simulink model "gtm_design"  (R2021b)
settings: Solver=VariableStepAuto  StartTime=0.0  StopTime=10.0  MinStep=0.00999  RelTol=1e-3
StopFcn:
  | MWSout=grabmws(bdroot);
  | MWSout.lastrun=datestr(now);
values from neighbouring files (symbols this model uses):
  knots2fps = 1.68781    [setup.m]
  s = tf('s')    [setup.m]
undefined symbols (not defined in the file or in its folder): Aero, aftfuel, aftfuel_pos, AILL, AILLC, AILR, AILRC, alpha_deg, alt0, altitude_ft, Ax_g, Ay_g, Az_g, b, beta_deg, bias, BRAKEC, Cbar, cg_pos0, cg_shift_gear, ControlMode, DamageCase, DamageModels, DamageOnsetTime, deltc, Earth, ELLIB, ELLIBC, ELLOB, ELLOBC, ELRIB, ELRIBC, ELROB, ELROBC, engl_ang, engl_pos, engr_ang, engr_pos, etas0, etas1, etasc_feedthrough, FLAPLC, FLAPLIB, FLAPLOB, FLAPRC, FLAPRIB, FLAPROB, FlightMode, FuelUsed_Init, fwdfuel, fwdfuel_pos, GEAR, GEARC, Inertia0, Inertia_shift_gear, Ixx_model, Iyy_model, Izz_model, KTAS, LandingGear ... (+66)
libraries: simulink_extras x98, LPVBlockLibrary x54, simulink_need_slupdate x30, aerolibconvert2 x27, simulink x7, aerolibtransform2 x6, uavalgslib x4, UserContent_lib x2, robotcorelib x1, uavutilslib x1
(part 2 of 9)

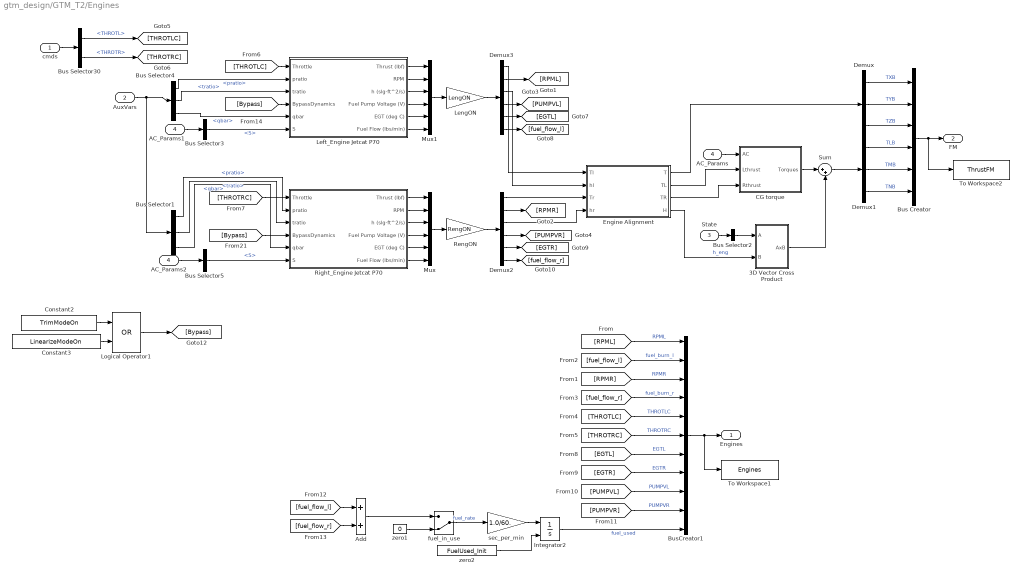
== system gtm_design/GTM_T2/Engines ==
  cmds : Inport
  AuxVars : Inport  Port=2
  State : Inport  Port=3
  AC_Params : Inport  Port=4
  3D Vector Cross Product : Subsystem
  AC_Params1 : InportShadow  Port=4
  AC_Params2 : InportShadow  Port=4
  Add : Sum
  Bus Creator : BusCreator  Inputs=6
  Bus Selector1 : BusSelector  OutputSignals=pratio,tratio,qbar
  Bus Selector2 : BusSelector  OutputSignals=pb,qb,rb  OutputAsBus=on
  Bus Selector3 : BusSelector  OutputSignals=S
  Bus Selector30 : BusSelector  OutputSignals=THROTL,THROTR
  Bus Selector4 : BusSelector  OutputSignals=pratio,tratio,qbar
  Bus Selector5 : BusSelector  OutputSignals=S
  BusCreator1 : BusCreator  Inputs=11
  CG torque : Subsystem
  Constant2 : Constant  Value=TrimModeOn
  Constant3 : Constant  Value=LinearizeModeOn
  Demux : Demux  Outputs=3
  Demux1 : Demux  Outputs=3
  Demux2 : Demux  Outputs=6
  Demux3 : Demux  Outputs=6
  Engine Alignment : MATLAB Function  TreatAsAtomicUnit=on
  Integrator2 : Integrator  InitialConditionSource=external
  Left_Engine Jetcat P70 : Subsystem
      mask init:
      | % Curve fit parameters for Jetcat P70 Model
      | % Coeff_thrust   = [0.000028864242464  -0.001914835880159 0.105916926095459  -1.251646340183624 ];
      | Coeff_thrust   = [0.000014847593013,  0, 0, 0.412662356277121];
      | Coeff_throttle = [0.000033035538475  -0.008354385314499 1.191126728328792 31.518959847101669];
      | Coeff_fuelflow = [0.000046800927870  -0.000779344124807 0.122178501497750];
      | Coeff_tau      = [ -2.2400e-02   2.9948e+00];
      | Coeff_EGT      = [ 2E-5, -0.0036,0.2342,-8.0496,664.99]; %EGT model, deg C
      | Coeff_dynamics = [ -.074 7.1];
      | fuelpump_table = [0 0.576	0.625	0.6985	0.7845	0.8575	0.919	0.9805	1.0415	1.1025...
      |                     1.1515	1.262	1.287	1.373	1.52	1.618	1.74	1.887	1.973...
      |                     2.12	2.255	2.4385	2.647	2.7575	2.9905	3.162]; %volts, table of fuel pump voltages
      | fuelflow_table = [0,0.0794,0.0876,0.102,0.1149,0.1275,0.1379,0.1487,0.1586,0.1671,...
      |                     0.1775,0.1858,0.194,0.2038,0.2206,0.2405,0.2566,0.2746,0.2921,0.3102,...
      |                     0.3266,0.3445,0.3533,0.3611,0.3866,0.4083;]*2; %lbs/min,   FULL fuel flow rates corresponding to pump voltages (fuelpump_table)  
      | % Equvalent Shaft parameters for engine
      | shaft_dia = 0.75/12.0;       % diameter of rotating turbine in feet 
      | shaft_len = 6.25/12.0;       % length of rotating turbine in feet   
      | density   = 15.2;            % mass density of steel in slugs/ft^3 
      | 
      | 
      | A = [-1.336,-0.7314;1,0;];
      | B = [1;0];
      | C = [-0.1474   0.7314];
      | D = 0;
  LengON : Gain  Gain=LengON  SaturateOnIntegerOverflow=on  OutDataTypeStr=Inherit: Same as input  ParamDataTypeStr=Inherit: Same as input
  Logical Operator1 : Logic  Operator=OR  AllPortsSameDT=off  OutDataTypeStr=boolean
  Mux : Mux  Inputs=6
  Mux1 : Mux  Inputs=6
  RengON : Gain  Gain=RengON  SaturateOnIntegerOverflow=on  OutDataTypeStr=Inherit: Same as input  ParamDataTypeStr=Inherit: Same as input
  Right_Engine Jetcat P70 : Subsystem
      mask init: same as gtm_design/GTM_T2/Engines/Left_Engine Jetcat P70
  Sum : Sum  Inputs=|++
  To Workspace1 : ToWorkspace  VariableName=Engines  SampleTime=-1
  To Workspace2 : ToWorkspace  VariableName=ThrustFM  SampleTime=-1
  fuel_in_use : ManualSwitch  CurrentSetting=0
  sec_per_min : Gain  Gain=1.0/60.  SaturateOnIntegerOverflow=on  OutDataTypeStr=Inherit: Same as input  ParamDataTypeStr=Inherit: Same as input
  zero1 : Constant  Value=0
  zero2 : Constant  Value=FuelUsed_Init
  Engines : Outport
  FM : Outport  Port=2  PortDimensions=6
  wires:
  cmds/1 -> Bus Selector30/1
  Demux/2 -> Bus Creator/2  "TYB"
  State/1 -> Bus Selector2/1
  Bus Selector2/1 -> 3D Vector Cross Product/1(A)
  Demux/3 -> Bus Creator/3  "TZB"
  AuxVars/1 -> Bus Selector1/1, Bus Selector4/1
  AC_Params/1 -> CG torque/1(AC)
  Bus Creator/1 -> To Workspace2/1, FM/1
  Bus Selector30/1 -> [THROTLC]  "<THROTL>"
  Bus Selector30/2 -> [THROTRC]  "<THROTR>"
  [THROTRC] -> BusCreator1/6  "THROTRC"
  [THROTLC] -> BusCreator1/5  "THROTLC"
  [fuel_flow_r] -> BusCreator1/4  "fuel_burn_r"
  [fuel_flow_l] -> BusCreator1/2  "fuel_burn_l"
  [RPMR] -> BusCreator1/3  "RPMR"
  [RPML] -> BusCreator1/1  "RPML"
  BusCreator1/1 -> To Workspace1/1, Engines/1
  [EGTL] -> BusCreator1/7  "EGTL"
  [EGTR] -> BusCreator1/8  "EGTR"
  [PUMPVL] -> BusCreator1/9  "PUMPVL"
  [PUMPVR] -> BusCreator1/10  "PUMPVR"
  sec_per_min/1 -> Integrator2/1
  fuel_in_use/1 -> sec_per_min/1  "fuel_rate"
  Integrator2/1 -> BusCreator1/11  "fuel_used"
  zero2/1 -> Integrator2/2
  [fuel_flow_l] -> Add/1
  [fuel_flow_r] -> Add/2
  zero1/1 -> fuel_in_use/2
  Add/1 -> fuel_in_use/1
  Demux/1 -> Bus Creator/1  "TXB"
  Engine Alignment/4(H) -> 3D Vector Cross Product/2(B)  "h_eng"
  Engine Alignment/1(T) -> Demux/1
  Engine Alignment/2(TL) -> CG torque/2(Lthrust)
  Engine Alignment/3(TR) -> CG torque/3(Rthrust)
  CG torque/1(Torques) -> Sum/1
  3D Vector Cross Product/1(AxB) -> Sum/2
  Sum/1 -> Demux1/1
  Demux1/1 -> Bus Creator/4  "TLB"
  Demux1/2 -> Bus Creator/5  "TMB"
  Demux1/3 -> Bus Creator/6  "TNB"
  Mux/1 -> RengON/1
  RengON/1 -> Demux2/1
  Demux2/1 -> Engine Alignment/3(Tr)
  Demux2/2 -> [RPMR]
  Demux2/3 -> Engine Alignment/4(hr)
  Demux2/4 -> [PUMPVR]
  Demux2/5 -> [EGTR]
  Demux2/6 -> [fuel_flow_r]
  Mux1/1 -> LengON/1
  LengON/1 -> Demux3/1
  Demux3/1 -> Engine Alignment/1(Tl)
  Demux3/2 -> [RPML]
  Demux3/3 -> Engine Alignment/2(hl)
  Demux3/4 -> [PUMPVL]
  Demux3/5 -> [EGTL]
  Demux3/6 -> [fuel_flow_l]
  Constant3/1 -> Logical Operator1/2
  Constant2/1 -> Logical Operator1/1
  Logical Operator1/1 -> [Bypass]
  Left_Engine Jetcat P70/1(Thrust (lbf)) -> Mux1/1
  Left_Engine Jetcat P70/2(RPM) -> Mux1/2
  Left_Engine Jetcat P70/3(h (slg-ft^2/s)) -> Mux1/3
  Left_Engine Jetcat P70/4(Fuel Pump Voltage (V)) -> Mux1/4
  Left_Engine Jetcat P70/5(EGT (deg C)) -> Mux1/5
  Left_Engine Jetcat P70/6(Fuel Flow (lbs/min)) -> Mux1/6
  Right_Engine Jetcat P70/1(Thrust (lbf)) -> Mux/1
  Right_Engine Jetcat P70/2(RPM) -> Mux/2
  Right_Engine Jetcat P70/3(h (slg-ft^2/s)) -> Mux/3
  Right_Engine Jetcat P70/4(Fuel Pump Voltage (V)) -> Mux/4
  Right_Engine Jetcat P70/5(EGT (deg C)) -> Mux/5
  Right_Engine Jetcat P70/6(Fuel Flow (lbs/min)) -> Mux/6
  AC_Params2/1 -> Bus Selector5/1
  AC_Params1/1 -> Bus Selector3/1
  [THROTRC] -> Right_Engine Jetcat P70/1(Throttle)
  Bus Selector4/1 -> Left_Engine Jetcat P70/2(pratio)  "<pratio>"
  Bus Selector4/2 -> Left_Engine Jetcat P70/3(tratio)  "<tratio>"
  [Bypass] -> Left_Engine Jetcat P70/4(BypassDynamics)
  Bus Selector4/3 -> Left_Engine Jetcat P70/5(qbar)  "<qbar>"
  Bus Selector3/1 -> Left_Engine Jetcat P70/6(S)  "<S>"
  Bus Selector1/1 -> Right_Engine Jetcat P70/2(pratio)  "<pratio>"
  Bus Selector1/2 -> Right_Engine Jetcat P70/3(tratio)  "<tratio>"
  [Bypass] -> Right_Engine Jetcat P70/4(BypassDynamics)
  Bus Selector1/3 -> Right_Engine Jetcat P70/5(qbar)  "<qbar>"
  Bus Selector5/1 -> Right_Engine Jetcat P70/6(S)  "<S>"
  [THROTLC] -> Left_Engine Jetcat P70/1(Throttle)

== system gtm_design/GTM_T2/Gravity ==
  AuxVars : Inport
  Params : Inport  Port=2
  Bus Selector1 : BusSelector  OutputSignals=DCM
  Bus Selector6 : BusSelector  OutputSignals=mass
  Ground : Ground
  Ground1 : Ground
  Mux : Mux  Inputs=[3 3]
  Mux1 : Mux  Inputs=3
  Product : Product  Multiplication=Matrix(*)  RndMeth=Zero
  Product1 : Product  RndMeth=Zero
  To Workspace2 : ToWorkspace  VariableName=GravityFM  SampleTime=-1
  acc due to gravity (ft/s^2) : Constant  Value=32.17405
  FM : Outport
  wires:
  acc due to gravity (ft/s^2)/1 -> Product1/2
  Ground1/1 -> Mux/2
  Product1/1 -> Mux1/3
  Ground/1 -> Mux1/2, Mux1/1
  Mux1/1 -> Product/2
  Mux/1 -> To Workspace2/1, FM/1
  Product/1 -> Mux/1
  Params/1 -> Bus Selector6/1
  AuxVars/1 -> Bus Selector1/1
  Bus Selector1/1 -> Product/1  "<DCM>"
  Bus Selector6/1 -> Product1/1  "<mass>"

== system gtm_design/GTM_T2/Landing Gear ==
  State : Inport
  Surfaces : Inport  Port=2
  ACParams : Inport  Port=3
  Bus Selector : BusSelector  OutputSignals=BRAKE,STEER,GEAR
  Bus Selector1 : BusSelector  OutputSignals=pb,qb,rb  OutputAsBus=on
  Bus Selector2 : BusSelector  OutputSignals=ub,vb,wb  OutputAsBus=on
  Bus Selector3 : BusSelector  OutputSignals=psi
  Bus Selector4 : BusSelector  OutputSignals=altitude
  Bus Selector5 : BusSelector  OutputSignals=phi,theta,psi  OutputAsBus=on
  Bus Selector6 : BusSelector  OutputSignals=CG  OutputAsBus=on
  Bus to Vector : BusToVector
  Bus to Vector1 : BusToVector
  Bus to Vector2 : BusToVector
  Gain : Gain  Gain=1/100
  LandingGear : Subsystem  mask{NoseWheelPos=LandingGear.NoseWheelPos, LeftMainPos=LandingGear.LeftMainPos, RightMainPos=LandingGear.RightMainPos, SpringConst=LandingGear.SpringConst, DampingConst=LandingGear.DampingConst, StrokeLength=LandingGear.StrokeLength, MountStiffness=LandingGear.MountStiff, MountDamping=LandingGear.MountDamping, RunwayAlt=runway_alt}
      mask prompts: NoseWheelPos "Nose Wheel Position [X,Y,Z]"; LeftMainPos "Left Main Position [X,Y,Z]"; RightMainPos "Right Main Position [X,Y,Z]"; SpringConst "Spring Constant [Nose,Left,Right]"; DampingConst "Damping Constant [Nose,Left,Right]"; StrokeLength "Stroke Length [Nose,Left,Right]"; MountStiffness "Mount Stiffness [Nose,Left,Right]"; MountDamping "Mount Damping [Nose,Left, Right]"; RunwayAlt "Runway Altitude"
      mask help:
      | Implements ground reaction force (if geardown is nonzero) for 3-wheel landing gear. Linear stiffness and damping are applied within stroke range, and (generally larger) mount stiffness and damping are applied beyond this range.
      |
      | Underlying gear.c function is from HL-20/LaRCsim, e.b.jackson@nasa.gov
  Mux : Mux  Inputs=2
  To Workspace1 : ToWorkspace  VariableName=GearState  SampleTime=-1
  To Workspace2 : ToWorkspace  VariableName=GearFM  SampleTime=-1
  FM : Outport
  GearState : Outport  Port=2
  wires:
  Mux/1 -> To Workspace2/1, FM/1
  Gain/1 -> LandingGear/7(Brake (0-1))
  LandingGear/3(Contact) -> To Workspace1/1, GearState/1
  LandingGear/2(M_gear) -> Mux/2
  LandingGear/1(F_gear) -> Mux/1
  Bus Selector/3 -> LandingGear/9(geardown (0/1))  "<GEAR>"
  Bus Selector/2 -> LandingGear/8(Steer (deg))  "<STEER>"
  Bus Selector/1 -> Gain/1  "<BRAKE>"
  Bus Selector3/1 -> LandingGear/6(Heading (Rad))  "<psi>"
  Bus to Vector/1 -> LandingGear/4(pqr (Rad/sec))
  Bus Selector4/1 -> LandingGear/3(Altitude (ft))  "<altitude>"
  Bus to Vector2/1 -> LandingGear/2(EulerAngles (Rad))
  Bus Selector6/1 -> LandingGear/1(cg)
  Surfaces/1 -> Bus Selector/1
  State/1 -> Bus Selector1/1, Bus Selector2/1, Bus Selector3/1, Bus Selector4/1, Bus Selector5/1
  Bus Selector1/1 -> Bus to Vector/1
  Bus to Vector1/1 -> LandingGear/5(Vbody (ft/sec))
  Bus Selector2/1 -> Bus to Vector1/1
  Bus Selector5/1 -> Bus to Vector2/1
  ACParams/1 -> Bus Selector6/1

== system gtm_design/GTM_T2/Sensors ==
  EOM_State : Inport
  EOM_Xdot : Inport  Port=2
  AC_Params : Inport  Port=3
  AuxVars : Inport  Port=4
  SurfacePos : Inport  Port=5
  Engines : Inport  Port=6
  Air Data : Subsystem
  AuxVars1 : InportShadow  Port=4
  Bus Creator : BusCreator  Inputs=5
  Engine ECU 8 Hz : Subsystem  SystemSampleTime=round(1/Timestep/8)*Timestep
  MAG3 IMU : Subsystem
  MIDG II 50 Hz : Subsystem  SystemSampleTime=round(1/Timestep/50)*Timestep
  Surface Pots : Subsystem
  Terminator : Terminator
  Terminator1 : Terminator
  To Workspace2 : ToWorkspace  VariableName=Sensors  SampleTime=-1
  Sensors : Outport
  wires:
  AC_Params/1 -> Terminator1/1
  EOM_Xdot/1 -> Terminator/1
  Bus Creator/1 -> To Workspace2/1, Sensors/1
  Air Data/1(AirData) -> Bus Creator/1  "AirData"
  MIDG II 50 Hz/1(MIDG) -> Bus Creator/2  "MIDG"
  Surface Pots/1(Pots) -> Bus Creator/4  "SurfacePos"
  Engine ECU 8 Hz/1(ECU) -> Bus Creator/5  "Engines"
  MAG3 IMU/1(MAG3) -> Bus Creator/3  "MAG3"
  Engines/1 -> Engine ECU 8 Hz/1(Engines)
  SurfacePos/1 -> Surface Pots/1(SurfacePos)
  AuxVars/1 -> Air Data/2(AuxVars), MIDG II 50 Hz/1(AuxVars)
  EOM_State/1 -> MIDG II 50 Hz/2(EOM_State), Air Data/1(EOM_State), MAG3 IMU/2(EOM_State)
  AuxVars1/1 -> MAG3 IMU/1(AuxVars)

== system gtm_design/GTM_T2/TransportDelay ==
  note: Uplink Path
  note: Downlink Path
  Sensors : Inport
  UL : Inport  Port=2
  AntiAliasing : Subsystem
  To Workspace2 : ToWorkspace  VariableName=DL  SampleTime=-1
  Transport Delay on Bus : Subsystem
  Transport Delay on Bus1 : Subsystem
  cmds : Outport
  DL : Outport  Port=2
  wires:
  AntiAliasing/1(O) -> Transport Delay on Bus/1(In)
  Transport Delay on Bus/1(Out) -> To Workspace2/1, DL/1
  UL/1 -> Transport Delay on Bus1/1(In)
  Sensors/1 -> AntiAliasing/1(I)
  Transport Delay on Bus1/1(Out) -> cmds/1

== system gtm_design/Guidance/Airspeed Step ==
  Action Port : ActionPort  ActionPortLabel=case [ 3 ]:
  Bus Creator : BusCreator  Inputs=5
  Constant1 : Constant  Value=-12.5
  Constant2 : Constant  Value=0
  Constant3 : Constant  Value=0
  Constant4 : Constant  Value=0
  Step : Step  Time=5  Before=80  After=90  SampleTime=0
  Step1 : Step  Commented=on  Time=50  After=-5  SampleTime=0
  Sum : Sum  Inputs=|++
  GuidanceCommand : Outport  InitialOutput=zeros(5,1)
  wires:
  Constant2/1 -> Bus Creator/2  "alt_c_ft"
  Constant4/1 -> Bus Creator/4  "phi_c_deg"
  Bus Creator/1 -> GuidanceCommand/1
  Constant3/1 -> Bus Creator/3  "bet_c_deg"
  Sum/1 -> Bus Creator/1  "tas_c_knot"
  Constant1/1 -> Bus Creator/5  "etas_c_percent"
  Step/1 -> Sum/1
  Step1/1 -> Sum/2

== system gtm_design/Guidance/Autopilot Step ==
  Action Port : ActionPort  ActionPortLabel=case [ 3 ]:
  Airspeed Step Command : Subsystem
  Altitude Step Command : Subsystem
  Constant : Constant  Value=3
  Gain : Gain  Gain=10
  GuidanceMode1 : Constant  Value=FlightMode
  Label : Subsystem
  Merge1 : Merge  Inputs=5
  Roll Angle Step Command : Subsystem
  Sideslip Step Command : Subsystem
  Sum : Sum  Inputs=|+-
  Switch Case1 : SwitchCase  CaseConditions={1,2,3,4}
  Zero : Subsystem
  round : Rounding  Operator=round
  cmd : Outport
  wires:
  Label/1(O) -> cmd/1
  Merge1/1 -> Label/1(I)
  Switch Case1/5 -> Zero/Action  "FlightMode == 3.0"
  Switch Case1/3 -> Sideslip Step Command/Action  "FlightMode == 3.3"
  Switch Case1/2 -> Altitude Step Command/Action  "FlightMode == 3.2"
  Switch Case1/1 -> Airspeed Step Command/Action  "FlightMode == 3.1"
  Sideslip Step Command/1(cmd) -> Merge1/3
  Airspeed Step Command/1(cmd) -> Merge1/1
  Altitude Step Command/1(cmd) -> Merge1/2
  Gain/1 -> round/1
  Sum/1 -> Gain/1
  Constant/1 -> Sum/2
  GuidanceMode1/1 -> Sum/1
  Roll Angle Step Command/1(cmd) -> Merge1/4
  Zero/1(cmd) -> Merge1/5
  Switch Case1/4 -> Roll Angle Step Command/Action  "FlightMode == 3.4"
  round/1 -> Switch Case1/1

== system gtm_design/Guidance/Autopilot Trajectory Tracking ==
  feedback : Inport
  Action Port : ActionPort  ActionPortLabel=case [ 4 ]:
  Constant : Constant  Value=4
  Constant1 : Constant  Value=4
  Constant2 : Constant  Value=2
  Gain : Gain  Gain=10
  Gain1 : Gain  Gain=10
  GuidanceMode1 : Constant  Value=FlightMode
  GuidanceMode2 : Constant  Value=FlightMode
  Label : Subsystem
  Orbit Following : Subsystem
  Sum : Sum  Inputs=|+-
  Sum1 : Sum  Inputs=|+-
  Sum2 : Sum  Inputs=|-+
  Switch : Switch  Criteria=u2 ~= 0
  Switch Case1 : SwitchCase  CaseConditions={1,2}  ShowDefaultCase=off
  Waypoint Following : Subsystem
  feedback1 : InportShadow
  round : Rounding  Operator=round
  round1 : Rounding  Operator=round
  guidance_cmd : Outport
  wires:
  Constant/1 -> Sum/2
  GuidanceMode1/1 -> Sum/1
  Waypoint Following/1(guidance_cmd) -> Switch/1
  Label/1(O) -> guidance_cmd/1
  Switch Case1/1 -> Waypoint Following/Action  "FlightMode == 4.1"
  Switch Case1/2 -> Orbit Following/Action  "FlightMode == 4.2"
  Sum/1 -> Gain/1
  Gain/1 -> round/1
  Orbit Following/1(guidance_cmd) -> Switch/3
  feedback/1 -> Waypoint Following/1(Feedback)
  feedback1/1 -> Orbit Following/1(Feedback)
  round/1 -> Switch Case1/1
  Sum1/1 -> Gain1/1
  GuidanceMode2/1 -> Sum1/1
  Gain1/1 -> round1/1
  Constant1/1 -> Sum1/2
  round1/1 -> Sum2/1
  Constant2/1 -> Sum2/2
  Sum2/1 -> Switch/2
  Switch/1 -> Label/1(I)

== system gtm_design/Guidance/CAS Maneuver ==
  Action Port : ActionPort  ActionPortLabel=case [ 2 ]:
  Constant : Constant  Value=2
  Gain : Gain  Gain=10
  GuidanceMode1 : Constant  Value=FlightMode
  High-g Turn : Subsystem
  Label : Subsystem
  Merge1 : Merge
  Push-over and Pull-up : Subsystem  Commented=on
  Sum : Sum  Inputs=|+-
  Switch Case1 : SwitchCase  CaseConditions={1,2}  ShowDefaultCase=off
  round : Rounding  Operator=round
  cmd : Outport
  wires:
  Label/1(O) -> cmd/1
  Merge1/1 -> Label/1(I)
  Switch Case1/2 -> High-g Turn/Action  "FlightMode == 2.2"
  Switch Case1/1 -> Push-over and Pull-up/Action  "FlightMode == 2.1"
  Gain/1 -> round/1
  Sum/1 -> Gain/1
  Constant/1 -> Sum/2
  GuidanceMode1/1 -> Sum/1
  Push-over and Pull-up/1(Out1) -> Merge1/1
  High-g Turn/1(Out1) -> Merge1/2
  round/1 -> Switch Case1/1

== system gtm_design/Guidance/CAS Step ==
  Action Port : ActionPort  ActionPortLabel=case [ 1 ]:
  Constant : Constant
  Gain : Gain  Gain=10
  GuidanceMode1 : Constant  Value=FlightMode
  Label : Subsystem
  Merge1 : Merge  Inputs=4
  Normal Acceleration Step Command : Subsystem
  Roll Rate Step Command : Subsystem
  Sideslip Step Command : Subsystem
  Sum : Sum  Inputs=|+-
  Switch Case1 : SwitchCase  CaseConditions={1,2,3}
  Zero : Subsystem
  round : Rounding  Operator=round
  cmd : Outport
  wires:
  GuidanceMode1/1 -> Sum/1
  Constant/1 -> Sum/2
  Sum/1 -> Gain/1
  Gain/1 -> round/1
  Sideslip Step Command/1(cmd) -> Merge1/2
  Normal Acceleration Step Command/1(cmd) -> Merge1/1
  Zero/1(cmd) -> Merge1/4
  Roll Rate Step Command/1(cmd) -> Merge1/3
  Switch Case1/1 -> Normal Acceleration Step Command/Action  "FlightMode == 1.1"
  Switch Case1/2 -> Sideslip Step Command/Action  "FlightMode == 1.2"
  Switch Case1/3 -> Roll Rate Step Command/Action  "FlightMode == 1.3"
  Switch Case1/4 -> Zero/Action  "FlightMode == 1.0"
  Merge1/1 -> Label/1(I)
  Label/1(O) -> cmd/1
  round/1 -> Switch Case1/1

== system gtm_design/Guidance/Elevation Step ==
  Action Port : ActionPort  ActionPortLabel=case [ 2 ]:
  Bus Creator : BusCreator  Inputs=5
  Constant : Constant  Value=80
  Constant1 : Constant  Value=-12.5
  Constant3 : Constant  Value=0
  Constant4 : Constant  Value=0
  Step : Step  After=10  SampleTime=0
  Step1 : Step  Commented=on  Time=50  After=-10  SampleTime=0
  Sum : Sum  Inputs=|++
  GuidanceCommand : Outport  InitialOutput=zeros(5,1)
  wires:
  Constant/1 -> Bus Creator/1  "tas_c_knot"
  Constant1/1 -> Bus Creator/5  "etas_c_percent"
  Constant3/1 -> Bus Creator/3  "bet_c_deg"
  Constant4/1 -> Bus Creator/4  "phi_c_deg"
  Bus Creator/1 -> GuidanceCommand/1
  Sum/1 -> Bus Creator/2  "alt_c_ft"
  Step1/1 -> Sum/2
  Step/1 -> Sum/1

== system gtm_design/Guidance/Heading Control ==
  guidance_cmd : Inport
  Feedback : Inport  Port=2
  Bus Creator1 : BusCreator  Inputs=7
  Bus Selector : BusSelector  OutputSignals=signal11
  Bus Selector1 : BusSelector  OutputSignals=alt_c_ft
  Constant1 : Constant  Value=tas0
  Constant3 : Constant  Value=0
  Constant4 : Constant  Value=0
  Constant5 : Constant  Value=etas0
  Constant6 : Constant
  FlightState : Subsystem
  Heading Control : MATLAB Function  TreatAsAtomicUnit=on  mask(Fixed Wing Heading Controller){PHeadingAngle=3.9}
      mask prompts: PHeadingAngle "Heading Control Gain"
      mask help: P controller that regulates fixed wing UAV heading direction through controlling its roll angle. This controller requires that the plane is flying under coordinated flight condition.
  Radians to Degrees : simulink_extras/Transformations/Radians to Degrees
  Saturation : Saturate  UpperLimit=phi_lim  LowerLimit=-phi_lim
  Windless : Subsystem  VariantControl=NoWind
      settings: PortSchema="{\"entries\":[{\"content\":{\"sides\":[{\"content\":{\"connectorIds\":[\"Out1\"]},\"type\":\"ConnectorPlacement.EquallySpacedRectSide\",\"uuid\":\"203a2d2a-30ae-46d5-b636-10933e29d1fa\"},{\"content\":{\"connectorIds\":[],\"side\":\"RIGHT\"},\"type\":\"ConnectorPlacement.EquallySpacedRectSide\",\"uuid\":\"332a648b-f7fb-47c3-be36-01d9c1955b3b\"},{\"content\":{\"connectorIds\":[],\"side\":\"TOP\"},\"type\":\"ConnectorPlacement.EquallySpacedRectSide\",\"uuid\":\"0294cf6c-fac0-4906-9702-b8e9ef362c1f\"}]},\"type\":\"ConnectorPlacement.EquallySpacedConnector\",\"uuid\":\"f608bdaf-466f-4a8f-9e8f-8d2734bc1053\"}],\"packageUris\":[\"http://schema.mathworks.com/mf0/Connector/R2020b\"],\"version\":\"1.0\"}"
  cmd : Outport
  wires:
  Radians to Degrees/1 -> Saturation/1
  Heading Control/1(RollAngle) -> Radians to Degrees/1  "phi_c_rad"
  Windless/1(Environment) -> Heading Control/3(e)
  Feedback/1 -> FlightState/1(Feedback)
  FlightState/1(FlightState) -> Heading Control/1(FlightState)  "FlightState"
  guidance_cmd/1 -> Bus Selector/1, Bus Selector1/1
  Bus Selector/1 -> Heading Control/2(UHeading)  "<signal11>"
  Bus Selector1/1 -> Bus Creator1/2  "<alt_c_ft>"
  Constant3/1 -> Bus Creator1/3  "bet_c_deg"
  Constant1/1 -> Bus Creator1/1  "tas_c_knot"
  Constant6/1 -> Bus Creator1/5  "an_c_g"
  Constant5/1 -> Bus Creator1/7  "etas_c_percent"
  Saturation/1 -> Bus Creator1/4  "phi_c_deg"
  Constant4/1 -> Bus Creator1/6  "p_c_deg"
  Bus Creator1/1 -> cmd/1

== system gtm_design/Guidance/Invalid, Error Out ==
  Action Port : ActionPort  ActionPortLabel=default:
  Constant1 : Constant  Value=zeros(5,1)
  Constant2 : Constant  Value=0
  InvalidMode : Assertion  AssertionFailFcn="warndlg('Invalid settings for TrimMode and LinearizeMode.  Run setup.m to reset.','Warning!')"
  Out : Outport  InitialOutput=zeros(5,1)
  wires:
  Constant1/1 -> Out/1
  Constant2/1 -> InvalidMode/1

== system gtm_design/Guidance/Label ==
  I : Inport
  I1 : Inport  Port=2
  Abs : Abs
  Add : Sum  Inputs=+++
  Bus Creator1 : BusCreator  Inputs=7
  Bus Selector : BusSelector  Commented=on  OutputSignals=AirData.KTAS,MIDG.NAV_altitude_m
  Demux1 : Demux  Outputs=7
  Gain : Gain  Gain=phi_to_eta
  Length Conversion : aerolibconvert2/Length Conversion  Commented=on  IU=m  OU=ft
  MATLAB Function : MATLAB Function  Commented=on  TreatAsAtomicUnit=on
  MATLAB Function1 : MATLAB Function  Commented=on  TreatAsAtomicUnit=on
  Ramp : simulink/Sources/Ramp  slope=RateofClimb  start=20  InitialOutput=0
  Ramp1 : simulink/Sources/Ramp  Commented=on  slope=0.1  start=0  InitialOutput=0
  Sum : Sum  Inputs=|++
  Sum1 : Sum  Inputs=|++
  Sum2 : Sum  Inputs=|++
  O : Outport
  wires:
  I/1 -> Demux1/1
  Sum/1 -> Bus Creator1/7  "etas_c_percent"
  Demux1/5 -> Bus Creator1/5  "an_c_g"
  Demux1/3 -> Bus Creator1/3  "bet_c_deg"
  Sum2/1 -> Bus Creator1/1  "tas_c_knot"
  Demux1/6 -> Bus Creator1/6  "p_c_deg"
  Sum1/1 -> Bus Creator1/2  "alt_c_ft"
  Demux1/4 -> Bus Creator1/4, Abs/1  "phi_c_deg"
  Bus Creator1/1 -> O/1
  Demux1/7 -> Sum/1  "etas_c_percent"
  Gain/1 -> Add/1
  Demux1/2 -> Sum1/1  "alt_c_ft"
  Ramp/1 -> Sum1/2
  Abs/1 -> Gain/1
  Demux1/1 -> Sum2/1  "tas_c_knot"
  Ramp1/1 -> Sum2/2
  MATLAB Function1/1(detas) -> Add/3
  MATLAB Function/1(detas) -> Add/2
  Add/1 -> Sum/2
  I1/1 -> Bus Selector/1
  Length Conversion/1 -> MATLAB Function1/1(alt_c_ft)
  Bus Selector/2 -> Length Conversion/1  "<NAV_altitude_m>"
  Bus Selector/1 -> MATLAB Function/1(tas_c_knot)  "<KTAS>"

== system gtm_design/Guidance/Level Flight ==
  Action Port : ActionPort  ActionPortLabel=case [ 1 ]:
  Bus Creator : BusCreator  Inputs=5
  Constant : Constant  Value=80
  Constant1 : Constant  Value=-12.5
  Constant2 : Constant  Value=0
  Constant3 : Constant  Value=0
  Constant4 : Constant  Value=0
  GuidanceCommand : Outport  InitialOutput=zeros(5,1)
  wires:
  Bus Creator/1 -> GuidanceCommand/1
  Constant3/1 -> Bus Creator/3  "bet_c_deg"
  Constant/1 -> Bus Creator/1  "tas_c_knot"
  Constant1/1 -> Bus Creator/5  "etas_c_percent"
  Constant4/1 -> Bus Creator/4  "phi_c_deg"
  Constant2/1 -> Bus Creator/2  "alt_c_ft"

== system gtm_design/Guidance/Orbit Following ==
  Feedback : Inport
  Action Port : ActionPort  ActionPortLabel=case [ 6 ]:
  Bus Creator : BusCreator  Inputs=5
  Bus Selector : BusSelector  OutputSignals=North,East,Height,HeadingAngle
  Constant : Constant  Value=80
  Constant1 : Constant  Value=-12.5
  Constant2 : Constant
  Constant3 : Constant  Value=0
  Constant4 : Constant  Value=1000
  Constant5 : Constant  Value=2000
  Gain2 : Gain  Gain=-1
  Gain5 : Gain  Gain=-1
  Heading Control : MATLAB Function  TreatAsAtomicUnit=on  mask(Fixed Wing Heading Controller){PHeadingAngle=1}
      mask prompts: PHeadingAngle "Heading Control Gain"
      mask help: P controller that regulates fixed wing UAV heading direction through controlling its roll angle. This controller requires that the plane is flying under coordinated flight condition.
  Length Conversion : aerolibconvert2/Length Conversion  IU=m  OU=ft
  Orbit Follower : uavalgslib/Orbit Follower  UAVType=fixed-wing  MinOrbitRadius=1  MinLookaheadDistance=0.1  ExternalReset=none  ShowCrossTrackErrorOutput=off  ShowNumTurnsOutput=off  SimulateUsing=Interpreted execution
      settings: SourceProductBaseCode=UV
  Radians to Degrees : simulink_extras/Transformations/Radians to Degrees
  Saturation1 : Saturate  UpperLimit=45  LowerLimit=-45
  Selector1 : Selector  InputPortWidth=3  IndexOptions=Index vector (dialog)  Indices=[3]  OutputSizes=1
  Signal Conversion : SignalConversion  OverrideOpt=off
  Signal Conversion1 : SignalConversion  OverrideOpt=off
  Subsystem1 : Subsystem
  Terminator3 : Terminator
  Terminator4 : Terminator
  Terminator5 : Terminator
  Vector Concatenate : Concatenate  NumInputs=4
  Waypoints1 : Constant  Value=[0;3500;0]  VectorParams1D=off
  Windless : Subsystem  VariantControl=NoWind
      settings: PortSchema="{\"entries\":[{\"content\":{\"sides\":[{\"content\":{\"connectorIds\":[\"Out1\"]},\"type\":\"ConnectorPlacement.EquallySpacedRectSide\",\"uuid\":\"203a2d2a-30ae-46d5-b636-10933e29d1fa\"},{\"content\":{\"connectorIds\":[],\"side\":\"RIGHT\"},\"type\":\"ConnectorPlacement.EquallySpacedRectSide\",\"uuid\":\"332a648b-f7fb-47c3-be36-01d9c1955b3b\"},{\"content\":{\"connectorIds\":[],\"side\":\"TOP\"},\"type\":\"ConnectorPlacement.EquallySpacedRectSide\",\"uuid\":\"0294cf6c-fac0-4906-9702-b8e9ef362c1f\"}]},\"type\":\"ConnectorPlacement.EquallySpacedConnector\",\"uuid\":\"f608bdaf-466f-4a8f-9e8f-8d2734bc1053\"}],\"packageUris\":[\"http://schema.mathworks.com/mf0/Connector/R2020b\"],\"version\":\"1.0\"}"
  GuidanceCommand : Outport  InitialOutput=zeros(5,1)
  LookaheadPoint : Outport  Port=2  InitialOutput=zeros(3,1)
  DesiredCourse : Outport  Port=3  InitialOutput=zeros(1,1)
  wires:
  Radians to Degrees/1 -> Saturation1/1
  Length Conversion/1 -> Bus Creator/2  "alt_c_ft"
  Saturation1/1 -> Bus Creator/4  "phi_c_deg"
  Constant5/1 -> Orbit Follower/3
  Selector1/1 -> Gain5/1
  Constant4/1 -> Orbit Follower/5
  Subsystem1/1(Out2) -> Heading Control/1(FlightState)  "FlightState"
  Constant2/1 -> Orbit Follower/4
  Gain5/1 -> Length Conversion/1  "Height"
  Constant1/1 -> Bus Creator/5  "etas_c_percent"
  Subsystem1/2(Out1) -> Bus Selector/1
  Waypoints1/1 -> Orbit Follower/2
  Orbit Follower/4 -> Terminator4/1
  Orbit Follower/3 -> Terminator3/1
  Heading Control/1(RollAngle) -> Radians to Degrees/1  "phi_c_rad"
  Orbit Follower/1 -> Signal Conversion/1, Selector1/1
  Orbit Follower/5 -> Terminator5/1
  Gain2/1 -> Vector Concatenate/3
  Constant/1 -> Bus Creator/1  "tas_c_knot"
  Windless/1(Environment) -> Heading Control/3(e)
  Constant3/1 -> Bus Creator/3  "bet_c_deg"
  Bus Selector/3 -> Gain2/1  "<Height>"
  Bus Selector/4 -> Vector Concatenate/4  "<HeadingAngle>"
  Bus Selector/1 -> Vector Concatenate/1  "<North>"
  Orbit Follower/2 -> Signal Conversion1/1, Heading Control/2(UHeading)
  Vector Concatenate/1 -> Orbit Follower/1
  Bus Selector/2 -> Vector Concatenate/2  "<East>"
  Bus Creator/1 -> GuidanceCommand/1
  Feedback/1 -> Subsystem1/1(Feedback)
  Signal Conversion/1 -> LookaheadPoint/1
  Signal Conversion1/1 -> DesiredCourse/1

== system gtm_design/Guidance/Roll Step ==
  Action Port : ActionPort  ActionPortLabel=case [ 4 ]:
  Bus Creator : BusCreator  Inputs=5
  Constant1 : Constant  Value=-12.5
  Constant2 : Constant  Value=0
  Constant4 : Constant  Value=0
  Constant5 : Constant  Value=80
  Step2 : Step  After=45  SampleTime=0
  GuidanceCommand : Outport  InitialOutput=zeros(5,1)
  wires:
  Constant1/1 -> Bus Creator/5  "etas_c_percent"
  Constant4/1 -> Bus Creator/3  "bet_c_deg"
  Constant2/1 -> Bus Creator/2  "alt_c_ft"
  Step2/1 -> Bus Creator/4  "phi_c_deg"
  Bus Creator/1 -> GuidanceCommand/1
  Constant5/1 -> Bus Creator/1  "tas_c_knot"

== system gtm_design/Guidance/Waypoint Following ==
  Feedback : Inport
  Action Port : ActionPort  ActionPortLabel=case [ 5 ]:
  Bus Creator : BusCreator  Inputs=5
  Bus Selector : BusSelector  OutputSignals=North,East,Height,HeadingAngle
  Constant : Constant  Value=80
  Constant1 : Constant  Value=-12.5
  Constant3 : Constant  Value=0
  Constant4 : Constant  Value=1000
  Gain2 : Gain  Gain=-1
  Gain5 : Gain  Gain=-1
  Heading Control : MATLAB Function  TreatAsAtomicUnit=on  mask(Fixed Wing Heading Controller){PHeadingAngle=3.9}
      mask prompts: PHeadingAngle "Heading Control Gain"
      mask help: P controller that regulates fixed wing UAV heading direction through controlling its roll angle. This controller requires that the plane is flying under coordinated flight condition.
  Length Conversion : aerolibconvert2/Length Conversion  IU=m  OU=ft
  Radians to Degrees : simulink_extras/Transformations/Radians to Degrees
  Saturation1 : Saturate  UpperLimit=30  LowerLimit=-30
  Selector1 : Selector  InputPortWidth=3  IndexOptions=Index vector (dialog)  Indices=[3]  OutputSizes=1
  Signal Conversion : SignalConversion  OverrideOpt=off
  Signal Conversion1 : SignalConversion  OverrideOpt=off
  Subsystem1 : Subsystem
  Terminator3 : Terminator
  Terminator4 : Terminator
  Vector Concatenate : Concatenate  NumInputs=4
  Waypoint Follower : uavalgslib/Waypoint Follower  UAVType=fixed-wing  StartFrom=first  TransitionRadiusSource=internal  TransitionRadius=100  MinLookaheadDistance=0.1  YawInput=off  ShowCrossTrackErrorOutput=off  ShowStatusOutput=off  SimulateUsing=Interpreted execution
      settings: SourceProductBaseCode=UV
  Waypoints : Constant  Value=[0;3000;0]  VectorParams1D=off
  Windless : Subsystem  VariantControl=NoWind
      settings: PortSchema="{\"entries\":[{\"content\":{\"sides\":[{\"content\":{\"connectorIds\":[\"Out1\"]},\"type\":\"ConnectorPlacement.EquallySpacedRectSide\",\"uuid\":\"203a2d2a-30ae-46d5-b636-10933e29d1fa\"},{\"content\":{\"connectorIds\":[],\"side\":\"RIGHT\"},\"type\":\"ConnectorPlacement.EquallySpacedRectSide\",\"uuid\":\"332a648b-f7fb-47c3-be36-01d9c1955b3b\"},{\"content\":{\"connectorIds\":[],\"side\":\"TOP\"},\"type\":\"ConnectorPlacement.EquallySpacedRectSide\",\"uuid\":\"0294cf6c-fac0-4906-9702-b8e9ef362c1f\"}]},\"type\":\"ConnectorPlacement.EquallySpacedConnector\",\"uuid\":\"f608bdaf-466f-4a8f-9e8f-8d2734bc1053\"}],\"packageUris\":[\"http://schema.mathworks.com/mf0/Connector/R2020b\"],\"version\":\"1.0\"}"
  GuidanceCommand : Outport  InitialOutput=zeros(5,1)
  LookaheadPoint : Outport  Port=2  InitialOutput=zeros(3,1)
  DesiredCourse : Outport  Port=3  InitialOutput=zeros(1,1)
  wires:
  Feedback/1 -> Subsystem1/1(Feedback)
  Bus Creator/1 -> GuidanceCommand/1
  Bus Selector/2 -> Vector Concatenate/2  "<East>"
  Vector Concatenate/1 -> Waypoint Follower/1
  Waypoint Follower/2 -> Signal Conversion1/1, Heading Control/2(UHeading)
  Bus Selector/1 -> Vector Concatenate/1  "<North>"
  Bus Selector/4 -> Vector Concatenate/4  "<HeadingAngle>"
  Bus Selector/3 -> Gain2/1  "<Height>"
  Constant3/1 -> Bus Creator/3  "bet_c_deg"
  Windless/1(Environment) -> Heading Control/3(e)
  Constant/1 -> Bus Creator/1  "tas_c_knot"
  Gain2/1 -> Vector Concatenate/3
  Waypoint Follower/1 -> Selector1/1, Signal Conversion/1
  Heading Control/1(RollAngle) -> Radians to Degrees/1  "phi_c_rad"
  Waypoint Follower/3 -> Terminator3/1
  Waypoint Follower/4 -> Terminator4/1
  Waypoints/1 -> Waypoint Follower/2
  Subsystem1/2(Out1) -> Bus Selector/1
  Constant1/1 -> Bus Creator/5  "etas_c_percent"
  Gain5/1 -> Length Conversion/1  "Height"
  Subsystem1/1(Out2) -> Heading Control/1(FlightState)  "FlightState"
  Constant4/1 -> Waypoint Follower/3
  Selector1/1 -> Gain5/1
  Saturation1/1 -> Bus Creator/4  "phi_c_deg"
  Length Conversion/1 -> Bus Creator/2  "alt_c_ft"
  Radians to Degrees/1 -> Saturation1/1
  Signal Conversion/1 -> LookaheadPoint/1
  Signal Conversion1/1 -> DesiredCourse/1

== system gtm_design/Control/BiasSurfs/Label ==
  In1 : Inport
  Bus Creator : BusCreator  Inputs=21
  Demux : Demux  Outputs=21
  UL : Outport
  wires:
  Demux/21 -> Bus Creator/21  "STEERC"
  Demux/19 -> Bus Creator/19  "GEARC"
  Demux/18 -> Bus Creator/18  "MORPHRC"
  Demux/2 -> Bus Creator/2  "THROTRC"
  Demux/6 -> Bus Creator/6  "ELRIBC"
  Demux/14 -> Bus Creator/14  "SPLROBC"
  Demux/7 -> Bus Creator/7  "AILLC"
  Demux/15 -> Bus Creator/15  "FLAPLC"
  Demux/10 -> Bus Creator/10  "RUDLOC"
  Demux/16 -> Bus Creator/16  "MORPHLC"
  Demux/12 -> Bus Creator/12  "SPLLOBC"
  Demux/9 -> Bus Creator/9  "RUDUPC"
  Bus Creator/1 -> UL/1
  Demux/11 -> Bus Creator/11  "SPLLIBC"
  In1/1 -> Demux/1
  Demux/13 -> Bus Creator/13  "SPLRIBC"
  Demux/1 -> Bus Creator/1  "THROTLC"
  Demux/5 -> Bus Creator/5  "ELROBC"
  Demux/8 -> Bus Creator/8  "AILRC"
  Demux/4 -> Bus Creator/4  "ELLIBC"
  Demux/20 -> Bus Creator/20  "BRAKEC"
  Demux/17 -> Bus Creator/17  "FLAPRC"
  Demux/3 -> Bus Creator/3  "ELLOBC"

== system gtm_design/Control/Controller/Bias Mixer ==
  In : Inport
  Elevator : Constant  Value=bias.elevator
  Flaps1 : Constant  Value=bias.rudder
  Flaps2 : Constant  Value=bias.aileron
  Flaps3 : Constant  Value=bias.morphing
  Flaps4 : Constant  Value=bias.morphing
  Mux : Mux  Inputs=6
  Sum : Sum  Inputs=|+-
  Throttle : Constant  Value=bias.throttle
  Out : Outport
  wires:
  Throttle/1 -> Mux/1
  Elevator/1 -> Mux/2
  Flaps2/1 -> Mux/3
  Flaps1/1 -> Mux/4
  Flaps3/1 -> Mux/5
  Flaps4/1 -> Mux/6
  In/1 -> Sum/1
  Mux/1 -> Sum/2
  Sum/1 -> Out/1

== system gtm_design/Control/Controller/Control Algorithm ==
  cmd : Inport
  feedback : Inport  Port=2
  Constant : Constant  Value=ControlMode
  Demux : Demux  Outputs=5
  Hinf Autopilot : Subsystem
  Hinf CAS : Subsystem
  LPV Autopilot : Subsystem
  LPV CAS : Subsystem
  Merge : Merge  Inputs=5  InitialOutput=zeros(5,1)
  No Control : Subsystem
  Switch Case : SwitchCase  CaseConditions={1,2,3,4}
  THROTC : Outport
  ELLC : Outport  Port=2
  AILC : Outport  Port=3
  RUDC : Outport  Port=4
  SPANAC : Outport  Port=5
  wires:
  Demux/5 -> SPANAC/1
  Demux/1 -> THROTC/1
  Demux/2 -> ELLC/1
  Demux/4 -> RUDC/1
  Demux/3 -> AILC/1
  cmd/1 -> [cmd]
  feedback/1 -> [feedback]
  [cmd] -> Hinf Autopilot/1(cmd)
  [feedback] -> Hinf Autopilot/2(feedback)
  [feedback] -> LPV CAS/2(feedback)
  [cmd] -> LPV CAS/1(cmd)
  [cmd] -> LPV Autopilot/1(cmd)
  [feedback] -> LPV Autopilot/2(feedback)
  Merge/1 -> Demux/1
  Constant/1 -> Switch Case/1
  [cmd] -> Hinf CAS/1(cmd)
  [feedback] -> Hinf CAS/2(feedback)
  Switch Case/5 -> No Control/Action
  Switch Case/4 -> LPV Autopilot/Action
  Switch Case/3 -> Hinf Autopilot/Action
  Switch Case/2 -> LPV CAS/Action
  Switch Case/1 -> Hinf CAS/Action
  Hinf CAS/1(CONTROLC) -> Merge/1
  LPV CAS/1(CONTROLC) -> Merge/2
  Hinf Autopilot/1(CONTROLC) -> Merge/3
  LPV Autopilot/1(CONTROLC) -> Merge/4
  No Control/1(CONTROLC) -> Merge/5

== system gtm_design/Control/Controller/Morphing Mixer ==
  SPANAC : Inport
  SPANSC : Inport  Port=2
  Add : Sum
  Constant : Constant  Value=etasc_feedthrough
  Sine Wave : Sin  Amplitude=12.5  Bias=-12.5  Frequency=0.5*2*pi  SampleTime=0
  Subtract : Sum  Inputs=+-
  Switch : Switch  Criteria=u2 ~= 0
  SPANLC : Outport
  SPANRC : Outport  Port=2
  wires:
  Switch/1 -> Subtract/1, Add/2
  SPANAC/1 -> Add/1, Subtract/2
  Subtract/1 -> SPANLC/1
  Add/1 -> SPANRC/1
  Constant/1 -> Switch/2
  SPANSC/1 -> Switch/1
  Sine Wave/1 -> Switch/3

== system gtm_design/GTM_T2/A//C parameters/Inertia//Mass//CG Shift ==
  note: Inertia "vector" = [Ixx Iyy Izz Ixz Iyz Ixy]
  gear : Inport
  fuel_used : Inport  Port=2
  DamageCase : Inport  Port=3
  morphing : Inport  Port=4
  Add : Sum
  Add1 : Sum  Inputs=+++++
  Add2 : Sum  Inputs=++++
  Add3 : Sum  Inputs=-+
  DamageEffects : Subsystem
  Divide1 : Product  Inputs=/*
  FuelBurnEffects : Subsystem
  Gain : Gain  Gain=1/32.17405
  MorphingEffects : Subsystem
  Reshape : Reshape
  Reshape1 : Reshape
  Switch : Switch  Threshold=0.5
  Switch1 : Switch  Threshold=0.5
  cg/weight : Subsystem
  "fuel cg shift, cg_pos0" : MATLAB Function  TreatAsAtomicUnit=on
  ixxb3 : Constant  Value=Inertia0
  ixxb7 : Constant  Value=w0
  xCG1 : Constant  Value=zeros(1,3)
  xCG3 : Constant  Value=Inertia_shift_gear
  xCG4 : Constant  Value=cg_shift_gear
  xCG5 : Constant  Value=zeros(1,6)
  Inertia : Outport
  mass : Outport  Port=2
  CG : Outport  Port=3
  wires:
  "fuel cg shift, cg_pos0"/1(y) -> Divide1/2
  Divide1/1 -> Add2/2
  Reshape1/1 -> Inertia/1
  Reshape/1 -> CG/1
  cg/weight/2(dweight) -> Add/1
  gear/1 -> Switch1/2, Switch/2
  cg/weight/1(dCG) -> Add2/1
  Add3/1 -> Add/2
  xCG1/1 -> Switch1/3
  xCG4/1 -> Switch1/1
  Switch1/1 -> Add2/3
  ixxb7/1 -> Add3/2
  Gain/1 -> mass/1
  Add2/1 -> Reshape/1
  Add/1 -> Divide1/1, Gain/1  "gwest"
  DamageCase/1 -> cg/weight/1(DamageCase), DamageEffects/1(In)
  DamageEffects/1(dInertia) -> Add1/3
  ixxb3/1 -> Add1/4
  fuel_used/1 -> "fuel cg shift, cg_pos0"/1(fuel_used), Add3/1, FuelBurnEffects/1(In)
  xCG5/1 -> Switch/3
  xCG3/1 -> Switch/1
  Add1/1 -> Reshape1/1
  Switch/1 -> Add1/1
  FuelBurnEffects/1(dInertia) -> Add1/2
  morphing/1 -> MorphingEffects/1(morphing)
  MorphingEffects/1(dInertia) -> Add1/5
  MorphingEffects/2(dCG) -> Add2/4

== system gtm_design/GTM_T2/A//C parameters/TriggerDamage ==
  Clock : Clock
  DamgeCase : Constant  Value=DamageCase
  Switch : Switch  Threshold=DamageOnsetTime
  Zero : Constant  Value=0
  damagecase : Outport
  wires:
  Clock/1 -> Switch/2
  Switch/1 -> damagecase/1
  Zero/1 -> Switch/3
  DamgeCase/1 -> Switch/1
